simulink model "Lab1Sim"  (R2025b)
settings: Solver=VariableStepAuto  StartTime=0.0  StopTime=50  RelTol=1e-3
values from neighbouring files (symbols this model uses):
  licznik = [1]    [Lab1.m]    (also in OG.m)
  mianownik = [30,11,1]    [Lab1.m]    (also in OG.m)
  sysd = c2d(sys, Tp, 'zoh')    [Lab1.m]
  Tp = 0.5    [Lab1.m]
undefined symbols (not defined in the file or in its folder): Ad, Bd, Cd, Dd
settings Model: Creator=dorian  LastModifiedBy=dorian

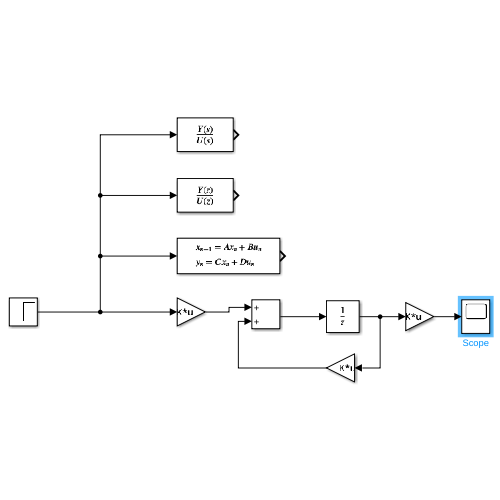
[thumbnail: Simulink's stored preview of the top-level diagram]
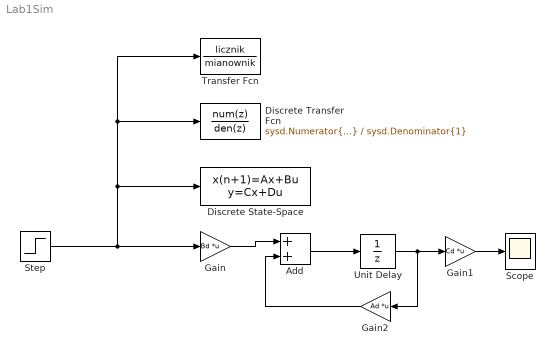
== system Lab1Sim ==
  Add : Sum
  Discrete Transfer Fcn : DiscreteTransferFcn  Numerator=sysd.Numerator{1}  Denominator=sysd.Denominator{1}  InitialStates=Tp
  Discrete State-Space : DiscreteStateSpace  A=Ad  B=Bd  C=Cd  D=Dd  SampleTime=-1
  Gain : Gain  Gain=Bd  Multiplication=Matrix(K*u)
  Gain1 : Gain  Gain=Cd  Multiplication=Matrix(K*u)
  Gain2 : Gain  Gain=Ad  Multiplication=Matrix(K*u)
  Scope : Scope
      settings: ActiveDisplayYMinimum=-0.11701571347436762  ActiveDisplayYMaximum=1.0531414212693089
  Step : Step  SampleTime=0
  Transfer Fcn : TransferFcn  Numerator=licznik  Denominator=mianownik
  Unit Delay : UnitDelay  SampleTime=-1  HasFrameUpgradeWarning=on
  wires:
  Step/1 -> Transfer Fcn/1, Discrete Transfer Fcn/1, Discrete State-Space/1, Gain/1
  Unit Delay/1 -> Gain2/1, Gain1/1
  Gain/1 -> Add/1
  Gain2/1 -> Add/2
  Add/1 -> Unit Delay/1
  Gain1/1 -> Scope/1
